simulink model "Digital_ACMC"  (R2026a)
settings: Solver=FixedStepAuto  StopTime=0.024  FixedStep=1e-8
undefined symbols (not defined in the file): Kbal, Ki_i, Ki_v, Kp_i, Kp_v, Vin
libraries: fl_lib x16, nesl_utility x11, ee_lib x4, eeGeneralControl x3, eePwmGenerator x2, simulink x1
settings Model: Creator=ardas  LastModifiedBy=ardas
settings SimscapeCC: SimscapeNominalValues="[{\"value\":\"1\",\"unit\":\"A\"},{\"value\":\"1\",\"unit\":\"bar\"},{\"value\":\"1\",\"unit\":\"cm^2\"},{\"value\":\"1\",\"unit\":\"cm^3/s\"},{\"value\":\"1\",\"unit\":\"kJ/kg\"},{\"value\":\"1\",\"unit\":\"kW\"},{\"value\":\"1\",\"unit\":\"l\"},{\"value\":\"1\",\"unit\":\"N\"},{\"value\":\"1\",\"unit\":\"N*m\"},{\"value\":\"1\",\"unit\":\"V\"}]"  SimscapeLogType=none  SimscapeLogDataHistory=5000.0

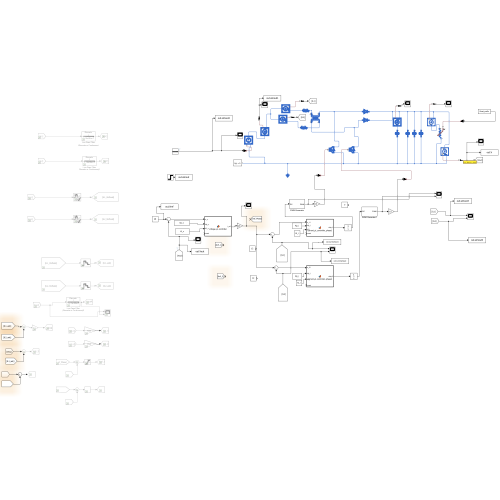
[thumbnail: Simulink's stored preview of the top-level diagram]
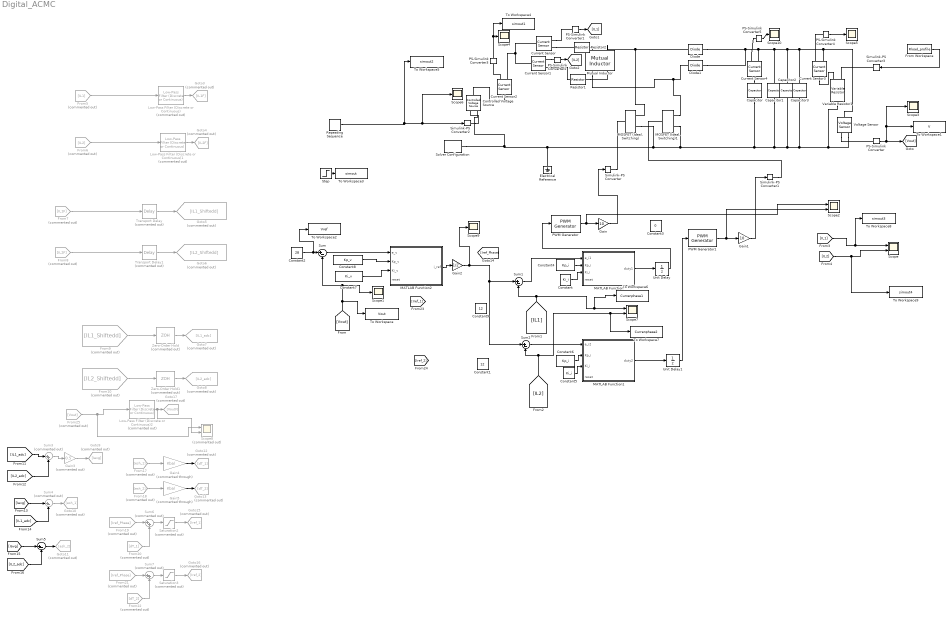
== system Digital_ACMC ==
  Capacitor : fl_lib/Electrical/Electrical Elements/Capacitor  c=330e-6 F  r=0.12 Ohm  g=0 1/Ohm  i_specify=off  i_priority=None  i=0 A  i_nominal_specify=off  i_nominal_value=1  i_nominal_unit=A  v_specify=off  v_priority=None  v=0 V  v_nominal_specify=off  v_nominal_value=1  v_nominal_unit=V  vc_specify=off  vc_priority=High  vc=0 V  vc_nominal_specify=off  vc_nominal_value=1  vc_nominal_unit=V
  Capacitor1 : fl_lib/Electrical/Electrical Elements/Capacitor  c=330e-6 F  r=0.12 Ohm  g=0 1/Ohm  i_specify=off  i_priority=None  i=0 A  i_nominal_specify=off  i_nominal_value=1  i_nominal_unit=A  v_specify=off  v_priority=None  v=0 V  v_nominal_specify=off  v_nominal_value=1  v_nominal_unit=V  vc_specify=off  vc_priority=High  vc=0 V  vc_nominal_specify=off  vc_nominal_value=1  vc_nominal_unit=V
  Capacitor2 : fl_lib/Electrical/Electrical Elements/Capacitor  c=47e-6 F  r=0.03 Ohm  g=0 1/Ohm  i_specify=off  i_priority=None  i=0 A  i_nominal_specify=off  i_nominal_value=1  i_nominal_unit=A  v_specify=off  v_priority=None  v=0 V  v_nominal_specify=off  v_nominal_value=1  v_nominal_unit=V  vc_specify=off  vc_priority=High  vc=0 V  vc_nominal_specify=off  vc_nominal_value=1  vc_nominal_unit=V
  Capacitor3 : fl_lib/Electrical/Electrical Elements/Capacitor  c=47e-6 F  r=0.03 Ohm  g=0 1/Ohm  i_specify=off  i_priority=None  i=0 A  i_nominal_specify=off  i_nominal_value=1  i_nominal_unit=A  v_specify=off  v_priority=None  v=0 V  v_nominal_specify=off  v_nominal_value=1  v_nominal_unit=V  vc_specify=off  vc_priority=High  vc=0 V  vc_nominal_specify=off  vc_nominal_value=1  vc_nominal_unit=V
  Constant : Constant  Value=Ki_i
  Constant1 : Constant  Value=12
  Constant2 : Constant  Value=28
  Constant3 : Constant  Value=0
  Constant4 : Constant  Value=Kp_i
  Constant5 : Constant  Value=Ki_i
  Constant6 : Constant  Value=Kp_i
  Constant7 : Constant  Value=Ki_v
  Constant8 : Constant  Value=Kp_v
  Constant9 : Constant  Value=12
  Controlled Voltage Source : fl_lib/Electrical/Electrical Sources/Controlled Voltage Source
  Current Sensor{,1..4} (5 alike) : fl_lib/Electrical/Electrical Sensors/Current Sensor
  Diode : ee_lib/Semiconductors & Converters/Diode  ModelType=ee.enum.diode.modelType.pwl  TableType=ee.enum.diode.tableType.IfMat  IfMat=[.07, .12, .19, 1.75, 4.24, 7.32, 11.2; .16, .3, .72, 2.14, 5.02, 8.35, 13.12] A  VfMat=[.9, 1.15, 1.25, 1.5, 1.75, 2.17, 2.6, 2.85; .58, .68, .75, 1.1, 1.38, 1.77, 2.27, 2.7] V  TjVec=[25, 125] degC  VfVec=[.5, .7, .9, 1.3, 1.7, 2.1, 2.5] V  IfVec=[.1, .2, .5, 1, 2, 4, 7, 10] A  IrMat=[1e-06, 2e-06, 5e-06, 1e-05, 2.5e-05, 5e-05, .0001; 2e-06, 5e-06, 1e-05, 4e-05, 8e-05, .0002, .0005] A  VrMat=[10, 100, 200, 250, 300, 325, 350; 10, 70, 160, 220, 270, 300, 320] V  VrVec=[10, 20, 40, 50, 70, 80, 100] V  IrVec=[1e-06, 2e-06, 5e-06, 1e-05, 2e-05, 5e-05, .0001] A  Vf=0.6 V  Ron=0.3 Ohm  Goff=1e-8 S  prmExp=ee.enum.diode.expParam.useTwo  I12=[.0137, .545] A  V12=[.6, .7] V  RS=0 Ohm  Tmeas=298.15 K  IS=1e-12 A  ec=1  I1=0.0137 A  V1=0.6 V  N_series=1  N_parallel=1  ZenerEnable=false  Rz=0.3 Ohm  BV=inf V  C_param=ee.enum.diode.capParam.fixed  CJ=0 pF  CJ0=5 pF  Vvec=[.1, 10, 100] V  Cvec=[3.5, 1, .4] pF  VJ=1 V  Mgrad=0.5  FC=0.5  Q_param=ee.enum.diode.recoveryParam.off  iRM=-7.15 A  iF=4 A  didt=-750 A/us  trr_factor=3  trr=115 ns  Qrr=150 nA*s  Vr=-600 V  Ls=150 nH  Erec=0.03 J  TT=50 ns  tau=100 ns  T_param=ee.enum.diode.temperatureParam.off  Tdevice=298.15 K  I1_T2=0.245 A  V1_T2=0.5 V  IS_T2=1.25e-7 A  Tmeas2=125 degC  XTI_param=ee.enum.diode.xtiParam.pn  XTI=3  EG_param=ee.enum.diode.egapParam.material_si  EG=1.11 eV  dBVdT=0 V/K  enable_fault_input=simscape.enum.onoff.off  i_specify=off  i_priority=None  i=0 A  i_nominal_specify=off  i_nominal_value=1  i_nominal_unit=A  v_specify=off  v_priority=None  v=0 V  v_nominal_specify=off  v_nominal_value=1  v_nominal_unit=V  v_capacitor_specify=off  v_capacitor_priority=None  v_capacitor=0 V  v_capacitor_nominal_specify=off  v_capacitor_nominal_value=1  v_capacitor_nominal_unit=V  Qj_specify=off  Qj_priority=High  Qj=0 C  Qj_nominal_specify=off  Qj_nominal_value=1  Qj_nominal_unit=C  i_diode_specify=off  i_diode_priority=None  i_diode=0 A  i_diode_nominal_specify=off  i_diode_nominal_value=1  i_diode_nominal_unit=A  v_diode_specify=off  v_diode_priority=None  v_diode=0 V  v_diode_nominal_specify=off  v_diode_nominal_value=1  v_diode_nominal_unit=V  i_capacitor_specify=off  i_capacitor_priority=None  i_capacitor=0 A  i_capacitor_nominal_specify=off  i_capacitor_nominal_value=1  i_capacitor_nominal_unit=A  fidelity_level=ee.enum.diode.fidelity.includeChargeDyn  rec_loss_model=ee.enum.diode.reverseRecoveryModel.fixed  ErecVal=0 J  scaleWithIandV=true  ErecMat=zeros(2, 3) J  ErecMat3D=zeros(2, 3, 2) J  TjrecVec=[298.15, 398.15] K  IfrecVec=[.1, 1, 10] A  IrecVal=10 A  VrecVal=10 V  VrecVec=[0, 100] V  tFilter=1 / 1000 / 100 s  thermal_network_parameterization=ee.enum.thermalNetworkTopology.junctionCase  Rth=[0, 10] K/W  Rth_Cauer=[1, 3, 10] K/W  Rth_Foster=[.08, .14, .22, .16] K/W  thermal_mass_parameterization=ee.enum.thermalNetwork.timeconstant  thermal_mass=[0, 1] J/K  thermal_mass_Cauer=[.1, .3, 1] J/K  thermal_mass_Foster=[.001, .005, .05, .5] J/K  thermal_time_constant=[0, 10] s  thermal_time_constant_Cauer=[1, 3, 10] s  thermal_time_constant_Foster=[7e-05, .0007, .01, .08] s  thermal_mass_initial_temperatures=[25, 25] degC  thermal_mass_initial_temperatures_Cauer=[25, 25, 25] degC  junction_thermal_mass=0.01 J/K  Tvec_initial_Foster=[25, 25, 25, 25] degC  no_thermal_network=0  junction_temperature_specify=off  junction_temperature_priority=None  junction_temperature=25 degC  junction_temperature_nominal_specify=off  junction_temperature_nominal_value=1  junction_temperature_nominal_unit=degC
  Diode1 : ee_lib/Semiconductors & Converters/Diode  ModelType=ee.enum.diode.modelType.pwl  TableType=ee.enum.diode.tableType.IfMat  IfMat=[.07, .12, .19, 1.75, 4.24, 7.32, 11.2; .16, .3, .72, 2.14, 5.02, 8.35, 13.12] A  VfMat=[.9, 1.15, 1.25, 1.5, 1.75, 2.17, 2.6, 2.85; .58, .68, .75, 1.1, 1.38, 1.77, 2.27, 2.7] V  TjVec=[25, 125] degC  VfVec=[.5, .7, .9, 1.3, 1.7, 2.1, 2.5] V  IfVec=[.1, .2, .5, 1, 2, 4, 7, 10] A  IrMat=[1e-06, 2e-06, 5e-06, 1e-05, 2.5e-05, 5e-05, .0001; 2e-06, 5e-06, 1e-05, 4e-05, 8e-05, .0002, .0005] A  VrMat=[10, 100, 200, 250, 300, 325, 350; 10, 70, 160, 220, 270, 300, 320] V  VrVec=[10, 20, 40, 50, 70, 80, 100] V  IrVec=[1e-06, 2e-06, 5e-06, 1e-05, 2e-05, 5e-05, .0001] A  Vf=0.6 V  Ron=0.3 Ohm  Goff=1e-8 S  prmExp=ee.enum.diode.expParam.useTwo  I12=[.0137, .545] A  V12=[.6, .7] V  RS=0 Ohm  Tmeas=298.15 K  IS=1e-12 A  ec=1  I1=0.0137 A  V1=0.6 V  N_series=1  N_parallel=1  ZenerEnable=false  Rz=0.3 Ohm  BV=inf V  C_param=ee.enum.diode.capParam.fixed  CJ=0 pF  CJ0=5 pF  Vvec=[.1, 10, 100] V  Cvec=[3.5, 1, .4] pF  VJ=1 V  Mgrad=0.5  FC=0.5  Q_param=ee.enum.diode.recoveryParam.off  iRM=-7.15 A  iF=4 A  didt=-750 A/us  trr_factor=3  trr=115 ns  Qrr=150 nA*s  Vr=-600 V  Ls=150 nH  Erec=0.03 J  TT=50 ns  tau=100 ns  T_param=ee.enum.diode.temperatureParam.off  Tdevice=298.15 K  I1_T2=0.245 A  V1_T2=0.5 V  IS_T2=1.25e-7 A  Tmeas2=125 degC  XTI_param=ee.enum.diode.xtiParam.pn  XTI=3  EG_param=ee.enum.diode.egapParam.material_si  EG=1.11 eV  dBVdT=0 V/K  enable_fault_input=simscape.enum.onoff.off  i_specify=off  i_priority=None  i=0 A  i_nominal_specify=off  i_nominal_value=1  i_nominal_unit=A  v_specify=off  v_priority=None  v=0 V  v_nominal_specify=off  v_nominal_value=1  v_nominal_unit=V  v_capacitor_specify=off  v_capacitor_priority=None  v_capacitor=0 V  v_capacitor_nominal_specify=off  v_capacitor_nominal_value=1  v_capacitor_nominal_unit=V  Qj_specify=off  Qj_priority=High  Qj=0 C  Qj_nominal_specify=off  Qj_nominal_value=1  Qj_nominal_unit=C  i_diode_specify=off  i_diode_priority=None  i_diode=0 A  i_diode_nominal_specify=off  i_diode_nominal_value=1  i_diode_nominal_unit=A  v_diode_specify=off  v_diode_priority=None  v_diode=0 V  v_diode_nominal_specify=off  v_diode_nominal_value=1  v_diode_nominal_unit=V  i_capacitor_specify=off  i_capacitor_priority=None  i_capacitor=0 A  i_capacitor_nominal_specify=off  i_capacitor_nominal_value=1  i_capacitor_nominal_unit=A  fidelity_level=ee.enum.diode.fidelity.includeChargeDyn  rec_loss_model=ee.enum.diode.reverseRecoveryModel.fixed  ErecVal=0 J  scaleWithIandV=true  ErecMat=zeros(2, 3) J  ErecMat3D=zeros(2, 3, 2) J  TjrecVec=[298.15, 398.15] K  IfrecVec=[.1, 1, 10] A  IrecVal=10 A  VrecVal=10 V  VrecVec=[0, 100] V  tFilter=1 / 1000 / 100 s  thermal_network_parameterization=ee.enum.thermalNetworkTopology.junctionCase  Rth=[0, 10] K/W  Rth_Cauer=[1, 3, 10] K/W  Rth_Foster=[.08, .14, .22, .16] K/W  thermal_mass_parameterization=ee.enum.thermalNetwork.timeconstant  thermal_mass=[0, 1] J/K  thermal_mass_Cauer=[.1, .3, 1] J/K  thermal_mass_Foster=[.001, .005, .05, .5] J/K  thermal_time_constant=[0, 10] s  thermal_time_constant_Cauer=[1, 3, 10] s  thermal_time_constant_Foster=[7e-05, .0007, .01, .08] s  thermal_mass_initial_temperatures=[25, 25] degC  thermal_mass_initial_temperatures_Cauer=[25, 25, 25] degC  junction_thermal_mass=0.01 J/K  Tvec_initial_Foster=[25, 25, 25, 25] degC  no_thermal_network=0  junction_temperature_specify=off  junction_temperature_priority=None  junction_temperature=25 degC  junction_temperature_nominal_specify=off  junction_temperature_nominal_value=1  junction_temperature_nominal_unit=degC
  Electrical Reference : fl_lib/Electrical/Electrical Elements/Electrical Reference
  From Workspace : FromWorkspace  VariableName=Rload_profile
  From10 : From  Commented=on  GotoTag=IL2_Shiftedd
  From17 : From  Commented=on  GotoTag=esh_1
  From18 : From  Commented=on  GotoTag=esh_2
  From19 : From  Commented=on  GotoTag=Iref_Phase
  From20 : From  Commented=on  GotoTag=dT_1
  From21 : From  Commented=on  GotoTag=Iref_Phase
  From22 : From  Commented=on  GotoTag=dT_2
  From25 : From  Commented=on  GotoTag=Vout
  From5 : From  Commented=on  GotoTag=IL1
  From6 : From  Commented=on  GotoTag=IL2
  From7 : From  Commented=on  GotoTag=IL1F
  From8 : From  Commented=on  GotoTag=IL2F
  From9 : From  Commented=on  GotoTag=IL1_Shiftedd
  Gain : Gain  Gain=10
  Gain1 : Gain  Gain=10
  Gain2 : Gain  Gain=1/2
  Gain3 : Gain  Commented=on  Gain=0.5
  Gain4 : Gain  Commented=through  Gain=Kbal
  Gain5 : Gain  Commented=through  Gain=Kbal
  Goto10 : Goto  Commented=on  GotoTag=esh_1
  Goto11 : Goto  Commented=on  GotoTag=esh_2
  Goto12 : Goto  Commented=on  GotoTag=dT_1
  Goto13 : Goto  Commented=on  GotoTag=dT_2
  Goto15 : Goto  Commented=on  GotoTag=Iref_1
  Goto16 : Goto  Commented=on  GotoTag=Iref_2
  Goto17 : Goto  Commented=on  GotoTag=VoutF
  Goto3 : Goto  Commented=on  GotoTag=IL1F
  Goto4 : Goto  Commented=on  GotoTag=IL2F
  Goto5 : Goto  Commented=on  GotoTag=IL1_Shiftedd
  Goto6 : Goto  Commented=on  GotoTag=IL2_Shiftedd
  Goto7 : Goto  Commented=on  GotoTag=IL1_adc
  Goto8 : Goto  Commented=on  GotoTag=IL2_adc
  Goto9 : Goto  Commented=on  GotoTag=Iavg
  Low-Pass Filter (Discrete or Continuous) : eeGeneralControl/Low-Pass Filter (Discrete or Continuous)  Commented=on  K=1  T=3.18e-5  B=inf  A=-inf  init_option=Inherited from block input  x0=0  Ts=-1
  Low-Pass Filter (Discrete or Continuous)1 : eeGeneralControl/Low-Pass Filter (Discrete or Continuous)  Commented=on  K=1  T=3.18e-5  B=inf  A=-inf  init_option=Inherited from block input  x0=0  Ts=-1
  Low-Pass Filter (Discrete or Continuous)2 : eeGeneralControl/Low-Pass Filter (Discrete or Continuous)  Commented=on  K=1  T=0.00003979  B=inf  A=-inf  init_option=Inherited from block input  x0=0  Ts=-1
  MATLAB Function : MATLAB Function  TreatAsAtomicUnit=on  SystemSampleTime=1e-5
  MATLAB Function1 : MATLAB Function  TreatAsAtomicUnit=on  SystemSampleTime=1e-5
  MATLAB Function2 : MATLAB Function  TreatAsAtomicUnit=on  SystemSampleTime=1e-4
  "MOSFET (Ideal, Switching)" : ee_lib/Semiconductors & Converters/MOSFET (Ideal, Switching)  port_option=ee.enum.controlport.ps  Rds=0.0028 Ohm  Goff=1e-6 1/Ohm  Vth=1.7 V  diode_param=ee.enum.semiconductors.protectionDiode.nodynamics  diode_Vf=0.83 V  diode_Ron=0.001 Ohm  diode_Goff=1e-5 1/Ohm  diode_C=50e-9 F  diode_iRM=-235 A  diode_iF=300 A  diode_idot=-50 A/us  diode_trr_param=ee.enum.converters.diodeReverseParam.trr_factor  diode_trr_factor=3  diode_trr=15 us  diode_Qrr=1500 s*uA  ids_specify=off  ids_priority=None  ids=0 A  ids_nominal_specify=off  ids_nominal_value=1  ids_nominal_unit=A  vds_specify=off  vds_priority=None  vds=0 V  vds_nominal_specify=off  vds_nominal_value=1  vds_nominal_unit=V  vgs_specify=off  vgs_priority=None  vgs=0 V  vgs_nominal_specify=off  vgs_nominal_value=1  vgs_nominal_unit=V  thermal_loss_option=ee.enum.converters.thermalLossOption.constantvalues  Von_data=[0, 1.8, 3.2, 6, 10, 16; 0, 2, 5.5, 9.5, 15, 25] V  Tj=[298.15, 448.15] K  Iout_data=[0, 20, 40, 60, 80, 100] A  tabulateWithVds=false  Eon_data=[0, 55.04, 124.57, 235.53, 362.12; 0, 71.25, 161.25, 304.88, 468.75] * 1e-6 J  Eoff_data=[0, 18, 30, 56.1, 76.5; 0, 22.5, 37.5, 70.13, 95.63] * 1e-6 J  Eon_data_3D=[zeros(2, 5, 3)] J  Eoff_data_3D=[zeros(2, 5, 3)] J  Tj_loss=[298.15, 448.15] K  Iout_data_loss=[0, 10, 20, 30, 40] A  Vds_loss=[0, 150, 300] V  Eon_scalar=22.86e-3 J  Eoff_scalar=17.14e-3 J  Voff=300 V  Iout_scalar=600 A  useCurrentFromPreviousCycle=false  useVoltageFromPreviousCycle=false  diodeModelType=ee.enum.converters.diodeModelType.pwl  diodeTableType=ee.enum.diode.tableType.IfMat  diode_ReverseIVType=ee.enum.diode.diodeReverseIV.constant  diode_IfMat=[.07, .12, .19, 1.75, 4.24, 7.32, 11.2; .16, .3, .72, 2.14, 4.02, 6.35, 9.12] A  diode_VfMat=[.9, 1.15, 1.25, 1.5, 1.75, 2.17, 2.6, 2.85; .58, .68, .75, 1.1, 1.38, 1.77, 2.27, 2.7] V  diode_TjVec=[25, 125] degC  diode_VfVec=[.5, .7, .9, 1.3, 1.7, 2.1, 2.5] V  diode_IfVec=[.1, .2, .5, 1, 2, 4, 7, 10] A  diode_IrMat=[1e-06, 2e-06, 5e-06, 1e-05, 2.5e-05, 5e-05, .0001; 2e-06, 5e-06, 1e-05, 4e-05, 8e-05, .0002, .0005] A  diode_VrMat=[10, 100, 200, 250, 300, 325, 350; 10, 70, 160, 220, 270, 300, 320] V  diode_VrVec=[10, 20, 40, 50, 70, 80, 100] V  diode_IrVec=[1e-06, 2e-06, 5e-06, 1e-05, 2e-05, 5e-05, .0001] A  diode_Vr=-600 V  diode_Ls=150 nH  diode_Erec=0.03 J  diode_rec_loss_model=ee.enum.diode.reverseRecoveryModel.fixed  diode_ErecVal=0 J  diode_scaleWithIandV=true  diode_ErecMat=zeros(2, 3) J  diodeErecMat3D=zeros(2, 3, 2) J  diode_TjrecVec=[298.15, 398.15] K  diode_IfrecVec=[.1, 1, 10] A  diodeVrecVec=[0, 100] V  diode_IrecVal=10 A  diode_VrecVal=10 V  diode_tFilter=1 / 1000 / 100 s  separateThermalPortForDiode=false  thermal_network_parameterization=ee.enum.thermalNetworkTopology.external  Rth=[.03, .2] K/W  Rth_Cauer=[.03, .1, .2] K/W  Rth_Foster=[.08, .14, .22, .16] K/W  thermal_mass_parameterization=ee.enum.thermalNetwork.timeconstant  thermal_mass=[3, 25] J/K  thermal_mass_Cauer=[3, 10, 25] J/K  thermal_mass_Foster=[.001, .005, .05, .5] J/K  thermal_time_constant=[.1, 5] s  thermal_time_constant_Cauer=[.1, 1, 5] s  thermal_time_constant_Foster=[7e-05, .0007, .01, .08] s  thermal_mass_initial_temperatures=[25, 25] degC  thermal_mass_initial_temperatures_Cauer=[25, 25, 25] degC  junction_thermal_mass=0.1 J/K  Tvec_initial_Foster=[25, 25, 25, 25] degC  RthDiode=[.03, .2] K/W  RthCauerDiode=[.03, .1, .2] K/W  RthFosterDiode=[.03, .2] K/W  thermalMassDiode=[3, 25] J/K  thermalMassCauerDiode=[3, 10, 25] J/K  thermalMassFosterDiode=[33, 50] J/K  thermalTauDiode=[.1, 5] s  thermalTauCauerDiode=[.1, 1, 5] s  thermalTauFosterDiode=[1, 10] s  thermalMassInitTempDiode=[25, 25] degC  thermalMassInitTempCauerDiode=[25, 25, 25] degC  junctionthermalMassDiode=0.1 J/K  TVecInitialFosterDiode=[25, 25, 25, 25] degC  no_thermal_network=0  mosfet_junction_temperature_specify=off  mosfet_junction_temperature_priority=None  mosfet_junction_temperature=25 degC  mosfet_junction_temperature_nominal_specify=off  mosfet_junction_temperature_nominal_value=1  mosfet_junction_temperature_nominal_unit=degC  diode_junction_temperature_specify=off  diode_junction_temperature_priority=None  diode_junction_temperature=25 degC  diode_junction_temperature_nominal_specify=off  diode_junction_temperature_nominal_value=1  diode_junction_temperature_nominal_unit=degC  Qj_specify=off  Qj_priority=None  Qj=0 W  Qj_nominal_specify=off  Qj_nominal_value=1  Qj_nominal_unit=W  accumulatedSwitchingLosses_specify=off  accumulatedSwitchingLosses_priority=None  accumulatedSwitchingLosses=0 J
  "MOSFET (Ideal, Switching)1" : ee_lib/Semiconductors & Converters/MOSFET (Ideal, Switching)  port_option=ee.enum.controlport.ps  Rds=0.0028 Ohm  Goff=1e-6 1/Ohm  Vth=1.7 V  diode_param=ee.enum.semiconductors.protectionDiode.nodynamics  diode_Vf=0.83 V  diode_Ron=0.001 Ohm  diode_Goff=1e-5 1/Ohm  diode_C=50e-9 F  diode_iRM=-235 A  diode_iF=300 A  diode_idot=-50 A/us  diode_trr_param=ee.enum.converters.diodeReverseParam.trr_factor  diode_trr_factor=3  diode_trr=15 us  diode_Qrr=1500 s*uA  ids_specify=off  ids_priority=None  ids=0 A  ids_nominal_specify=off  ids_nominal_value=1  ids_nominal_unit=A  vds_specify=off  vds_priority=None  vds=0 V  vds_nominal_specify=off  vds_nominal_value=1  vds_nominal_unit=V  vgs_specify=off  vgs_priority=None  vgs=0 V  vgs_nominal_specify=off  vgs_nominal_value=1  vgs_nominal_unit=V  thermal_loss_option=ee.enum.converters.thermalLossOption.constantvalues  Von_data=[0, 1.8, 3.2, 6, 10, 16; 0, 2, 5.5, 9.5, 15, 25] V  Tj=[298.15, 448.15] K  Iout_data=[0, 20, 40, 60, 80, 100] A  tabulateWithVds=false  Eon_data=[0, 55.04, 124.57, 235.53, 362.12; 0, 71.25, 161.25, 304.88, 468.75] * 1e-6 J  Eoff_data=[0, 18, 30, 56.1, 76.5; 0, 22.5, 37.5, 70.13, 95.63] * 1e-6 J  Eon_data_3D=[zeros(2, 5, 3)] J  Eoff_data_3D=[zeros(2, 5, 3)] J  Tj_loss=[298.15, 448.15] K  Iout_data_loss=[0, 10, 20, 30, 40] A  Vds_loss=[0, 150, 300] V  Eon_scalar=22.86e-3 J  Eoff_scalar=17.14e-3 J  Voff=300 V  Iout_scalar=600 A  useCurrentFromPreviousCycle=false  useVoltageFromPreviousCycle=false  diodeModelType=ee.enum.converters.diodeModelType.pwl  diodeTableType=ee.enum.diode.tableType.IfMat  diode_ReverseIVType=ee.enum.diode.diodeReverseIV.constant  diode_IfMat=[.07, .12, .19, 1.75, 4.24, 7.32, 11.2; .16, .3, .72, 2.14, 4.02, 6.35, 9.12] A  diode_VfMat=[.9, 1.15, 1.25, 1.5, 1.75, 2.17, 2.6, 2.85; .58, .68, .75, 1.1, 1.38, 1.77, 2.27, 2.7] V  diode_TjVec=[25, 125] degC  diode_VfVec=[.5, .7, .9, 1.3, 1.7, 2.1, 2.5] V  diode_IfVec=[.1, .2, .5, 1, 2, 4, 7, 10] A  diode_IrMat=[1e-06, 2e-06, 5e-06, 1e-05, 2.5e-05, 5e-05, .0001; 2e-06, 5e-06, 1e-05, 4e-05, 8e-05, .0002, .0005] A  diode_VrMat=[10, 100, 200, 250, 300, 325, 350; 10, 70, 160, 220, 270, 300, 320] V  diode_VrVec=[10, 20, 40, 50, 70, 80, 100] V  diode_IrVec=[1e-06, 2e-06, 5e-06, 1e-05, 2e-05, 5e-05, .0001] A  diode_Vr=-600 V  diode_Ls=150 nH  diode_Erec=0.03 J  diode_rec_loss_model=ee.enum.diode.reverseRecoveryModel.fixed  diode_ErecVal=0 J  diode_scaleWithIandV=true  diode_ErecMat=zeros(2, 3) J  diodeErecMat3D=zeros(2, 3, 2) J  diode_TjrecVec=[298.15, 398.15] K  diode_IfrecVec=[.1, 1, 10] A  diodeVrecVec=[0, 100] V  diode_IrecVal=10 A  diode_VrecVal=10 V  diode_tFilter=1 / 1000 / 100 s  separateThermalPortForDiode=false  thermal_network_parameterization=ee.enum.thermalNetworkTopology.external  Rth=[.03, .2] K/W  Rth_Cauer=[.03, .1, .2] K/W  Rth_Foster=[.08, .14, .22, .16] K/W  thermal_mass_parameterization=ee.enum.thermalNetwork.timeconstant  thermal_mass=[3, 25] J/K  thermal_mass_Cauer=[3, 10, 25] J/K  thermal_mass_Foster=[.001, .005, .05, .5] J/K  thermal_time_constant=[.1, 5] s  thermal_time_constant_Cauer=[.1, 1, 5] s  thermal_time_constant_Foster=[7e-05, .0007, .01, .08] s  thermal_mass_initial_temperatures=[25, 25] degC  thermal_mass_initial_temperatures_Cauer=[25, 25, 25] degC  junction_thermal_mass=0.1 J/K  Tvec_initial_Foster=[25, 25, 25, 25] degC  RthDiode=[.03, .2] K/W  RthCauerDiode=[.03, .1, .2] K/W  RthFosterDiode=[.03, .2] K/W  thermalMassDiode=[3, 25] J/K  thermalMassCauerDiode=[3, 10, 25] J/K  thermalMassFosterDiode=[33, 50] J/K  thermalTauDiode=[.1, 5] s  thermalTauCauerDiode=[.1, 1, 5] s  thermalTauFosterDiode=[1, 10] s  thermalMassInitTempDiode=[25, 25] degC  thermalMassInitTempCauerDiode=[25, 25, 25] degC  junctionthermalMassDiode=0.1 J/K  TVecInitialFosterDiode=[25, 25, 25, 25] degC  no_thermal_network=0  mosfet_junction_temperature_specify=off  mosfet_junction_temperature_priority=None  mosfet_junction_temperature=25 degC  mosfet_junction_temperature_nominal_specify=off  mosfet_junction_temperature_nominal_value=1  mosfet_junction_temperature_nominal_unit=degC  diode_junction_temperature_specify=off  diode_junction_temperature_priority=None  diode_junction_temperature=25 degC  diode_junction_temperature_nominal_specify=off  diode_junction_temperature_nominal_value=1  diode_junction_temperature_nominal_unit=degC  Qj_specify=off  Qj_priority=None  Qj=0 W  Qj_nominal_specify=off  Qj_nominal_value=1  Qj_nominal_unit=W  accumulatedSwitchingLosses_specify=off  accumulatedSwitchingLosses_priority=None  accumulatedSwitchingLosses=0 J
  Mutual Inductor : fl_lib/Electrical/Electrical Elements/Mutual Inductor  L1=120 uH  L2=120 uH  perfectCoupling=false  k=0.7  i1_specify=off  i1_priority=None  i1=0 A  i1_nominal_specify=off  i1_nominal_value=1  i1_nominal_unit=A  i2_specify=off  i2_priority=None  i2=0 A  i2_nominal_specify=off  i2_nominal_value=1  i2_nominal_unit=A  v1_specify=off  v1_priority=None  v1=0 V  v1_nominal_specify=off  v1_nominal_value=1  v1_nominal_unit=V  v2_specify=off  v2_priority=None  v2=0 V  v2_nominal_specify=off  v2_nominal_value=1  v2_nominal_unit=V
  PS-Simulink Converter : nesl_utility/PS-Simulink Converter  PhysicalDomain=network_engine_domain  SubClassName=ps_output  LeftPortType=input  RightPortType=output  PseudoPeriodic=off  Frequencies=[]  VectorFormat=inherit  Unit=V  AffineConversion=off
  PS-Simulink Converter1 : nesl_utility/PS-Simulink Converter  PhysicalDomain=network_engine_domain  SubClassName=ps_output  LeftPortType=input  RightPortType=output  PseudoPeriodic=off  Frequencies=[]  VectorFormat=inherit  Unit=A  AffineConversion=off
  PS-Simulink Converter2 : nesl_utility/PS-Simulink Converter  PhysicalDomain=network_engine_domain  SubClassName=ps_output  LeftPortType=input  RightPortType=output  PseudoPeriodic=off  Frequencies=[]  VectorFormat=inherit  Unit=A  AffineConversion=off
  PS-Simulink Converter3 : nesl_utility/PS-Simulink Converter  PhysicalDomain=network_engine_domain  SubClassName=ps_output  LeftPortType=input  RightPortType=output  PseudoPeriodic=off  Frequencies=[]  VectorFormat=inherit  Unit=inherit  AffineConversion=off
  PS-Simulink Converter4 : nesl_utility/PS-Simulink Converter  PhysicalDomain=network_engine_domain  SubClassName=ps_output  LeftPortType=input  RightPortType=output  PseudoPeriodic=off  Frequencies=[]  VectorFormat=inherit  Unit=inherit  AffineConversion=off
  PS-Simulink Converter5 : nesl_utility/PS-Simulink Converter  PhysicalDomain=network_engine_domain  SubClassName=ps_output  LeftPortType=input  RightPortType=output  PseudoPeriodic=off  Frequencies=[]  VectorFormat=inherit  Unit=inherit  AffineConversion=off
  PWM Generator : eePwmGenerator/PWM Generator  CarrCount=Up  Tper=10e-6  Tdelay=0  Ts=0.00000001
  PWM Generator1 : eePwmGenerator/PWM Generator  CarrCount=Up  Tper=10e-6  Tdelay=10e-6/2  Ts=0.00000001
  Repeating Sequence : simulink/Sources/Repeating Sequence  rep_seq_t="[0  6e-3 12e-3 18e-3 24e-3 ]"  rep_seq_y=[Vin Vin Vin Vin Vin]
  Resistor1 : fl_lib/Electrical/Electrical Elements/Resistor  R=0.01 Ohm  i_specify=off  i_priority=None  i=0 A  i_nominal_specify=off  i_nominal_value=1  i_nominal_unit=A  v_specify=off  v_priority=None  v=0 V  v_nominal_specify=off  v_nominal_value=1  v_nominal_unit=V
  Resistor2 : fl_lib/Electrical/Electrical Elements/Resistor  R=0.01 Ohm  i_specify=off  i_priority=None  i=0 A  i_nominal_specify=off  i_nominal_value=1  i_nominal_unit=A  v_specify=off  v_priority=None  v=0 V  v_nominal_specify=off  v_nominal_value=1  v_nominal_unit=V
  Saturation2 : Saturate  Commented=on  UpperLimit=15
  Saturation3 : Saturate  Commented=on  UpperLimit=15
  Scope : Scope  NumInputPorts=2
      settings: ActiveDisplayYMinimum=13.12118877178229  ActiveDisplayYMaximum=16.285901492217782
  Scope{1,3..6,9..10} (7 alike) : Scope
      Scope1 settings: ActiveDisplayYMinimum=27.996735188156986  ActiveDisplayYMaximum=28.000584839765885
      Scope10 settings: ActiveDisplayYMinimum=-21.021061924806343  ActiveDisplayYMaximum=8.27266243165029  DataLoggingVariableName=ScopeData10
      Scope3 settings: ActiveDisplayYMinimum=-3.5667585387126168  ActiveDisplayYMaximum=32.100857060330128  DataLoggingVariableName=ScopeData3
      Scope4 settings: ActiveDisplayYMinimum=25.497706773431442  ActiveDisplayYMaximum=29.783336297580011  DataLoggingVariableName=ScopeData4
      Scope5 settings: ActiveDisplayYMinimum=-12.32466223431901  ActiveDisplayYMaximum=-10.00882655979523  DataLoggingVariableName=ScopeData5
      Scope6 settings: ActiveDisplayYMinimum=10  ActiveDisplayYMaximum=30  DataLoggingVariableName=ScopeData6
      Scope9 settings: ActiveDisplayYMinimum=9.4576280676363549  ActiveDisplayYMaximum=13.640782053911529  DataLoggingVariableName=ScopeData9
  Scope2 : Scope  NumInputPorts=2
      settings: ActiveDisplayYMinimum=-0.05013738001407067  ActiveDisplayYMaximum=1.1748487112641266  DataLoggingVariableName=ScopeData2
  Scope7 : Scope  NumInputPorts=2
      settings: ActiveDisplayYMinimum=13.787058146219982  ActiveDisplayYMaximum=13.928836276625423  DataLoggingVariableName=ScopeData7
  Scope8 : Scope  Commented=on  NumInputPorts=2
      settings: ActiveDisplayYMinimum=5.4638907833296742  ActiveDisplayYMaximum=25.7507092946611  DataLoggingVariableName=ScopeData8
  Simulink-PS Converter : nesl_utility/Simulink-PS Converter  PhysicalDomain=network_engine_domain  SubClassName=ps_input  LeftPortType=input  RightPortType=output  PseudoPeriodic=off  Frequencies=[]  NoiseDistribution=none  NoiseParameters=[]  Unit=1  AffineConversion=off  FilteringAndDerivatives=provide  SimscapeFilterOrder=1  InputFilterTimeConstant=0.001  UdotUserProvided=0
  Simulink-PS Converter1 : nesl_utility/Simulink-PS Converter  PhysicalDomain=network_engine_domain  SubClassName=ps_input  LeftPortType=input  RightPortType=output  PseudoPeriodic=off  Frequencies=[]  NoiseDistribution=none  NoiseParameters=[]  Unit=1  AffineConversion=off  FilteringAndDerivatives=provide  SimscapeFilterOrder=1  InputFilterTimeConstant=0.001  UdotUserProvided=0
  Simulink-PS Converter2 : nesl_utility/Simulink-PS Converter  PhysicalDomain=network_engine_domain  SubClassName=ps_input  LeftPortType=input  RightPortType=output  PseudoPeriodic=off  Frequencies=[]  NoiseDistribution=none  NoiseParameters=[]  Unit=1  AffineConversion=off  FilteringAndDerivatives=provide  SimscapeFilterOrder=1  InputFilterTimeConstant=0.001  UdotUserProvided=0
  Simulink-PS Converter3 : nesl_utility/Simulink-PS Converter  PhysicalDomain=network_engine_domain  SubClassName=ps_input  LeftPortType=input  RightPortType=output  PseudoPeriodic=off  Frequencies=[]  NoiseDistribution=none  NoiseParameters=[]  Unit=Ohm  AffineConversion=off  FilteringAndDerivatives=provide  SimscapeFilterOrder=1  InputFilterTimeConstant=0.001  UdotUserProvided=0
  Solver Configuration : nesl_utility/Solver Configuration  PhysicalDomain=network_engine_domain  SubClassName=solver  LeftPortType=input  RightPortType=generic  Tones=[]  Harmonics=[]  SimulateNoise=off  Profile=off  UseLocalSampling=off  EnableSwitchedLinearOptims=on  FrequencyDomain=off  UseCCode=off  RelTol=0.001  AbsTol=0.001  MinStep=1e-09  ToWorkspace=off  RevertToSquareIcSolve=off  NumHomotopyIterations=100  PhasorMode=off  PhasorModeNumHarmonics=1  ConsistencySolver=NEWTON_XTOL_AFTER_FTOL  CanonicalOrdering=UNORDERED  OptimizeIntermediates=UNOPTIMIZED  IndexReductionMethod=DerivativeReplacement  DoDC=off  ResidualTolerance=1e-09  ConsistencyTolSource=GLOBAL  ConsistencyAbsTol=0.001  ConsistencyRelTol=0.001  ConsistencyTolFactor=0.001  UseLocalSolver=off  LocalSolverChoice=NE_BACKWARD_EULER_ADVANCER  ResolveIndetEquations=on  FunctionEvalNumThread=1  LocalSolverSampleTime=0.001  DoFixedCost=off  MaxNonlinIter=3  MaxModeIter=2  ComputeImpulses=off  ImpulseIterations=2  LinearAlgebra=auto  LinearAlgebraNumThread=0  EquationFormulation=NE_TIME_EF  DelaysMemoryBudget=1024  AutomaticFiltering=on  FilteringTimeConstant=0.001  PartitionStorageMethod=AS_NEEDED  PartitionMemoryBudget=1024  PartitionMethod=ROBUST  MultibodyUseLocalSolver=off  MultibodyLocalSolverChoice=ODE1  MultibodyLocalSolverSampleTime=0.001
  Step : Step  Time=0  FinalValue=28  SampleTime=0
  Sum{,1..2,5} (4 alike) : Sum  Inputs=|+-
  Sum3 : Sum  Commented=on  Inputs=|++
  Sum4 : Sum  Commented=on  Inputs=|+-
  Sum6 : Sum  Commented=on  Inputs=|++
  Sum7 : Sum  Commented=on  Inputs=|++
  To Workspace : ToWorkspace  VariableName=Vout  SaveFormat=Timeseries  SampleTime=-1
  To Workspace1 : ToWorkspace  VariableName=V  SaveFormat=Timeseries  SampleTime=-1
  To Workspace2 : ToWorkspace  VariableName=Vref  SaveFormat=Timeseries  SampleTime=-1
  To Workspace3 : ToWorkspace  VariableName=simout  SaveFormat=Timeseries  SampleTime=-1
  To Workspace4 : ToWorkspace  VariableName=simout1  SaveFormat=Timeseries  SampleTime=-1
  To Workspace5 : ToWorkspace  VariableName=simout2  SaveFormat=Timeseries  SampleTime=-1
  To Workspace6 : ToWorkspace  VariableName=Currenphase1  SaveFormat=Timeseries  SampleTime=-1
  To Workspace7 : ToWorkspace  VariableName=Currenphase2  SaveFormat=Timeseries  SampleTime=-1
  To Workspace8 : ToWorkspace  VariableName=simout3  SaveFormat=Timeseries  SampleTime=-1
  To Workspace9 : ToWorkspace  VariableName=simout4  SaveFormat=Timeseries  SampleTime=-1
  Transport Delay : TransportDelay  Commented=on  DelayTime=5e-6
  Transport Delay1 : TransportDelay  Commented=on  DelayTime=5e-6
  Unit Delay : UnitDelay  SampleTime=-1
  Unit Delay1 : UnitDelay  SampleTime=-1
  Variable Resistor1 : fl_lib/Electrical/Electrical Elements/Variable Resistor  Rmin=0 Ohm  thermalEnable=false  thermal_mass=1 J/K  i_specify=off  i_priority=None  i=0 A  i_nominal_specify=off  i_nominal_value=1  i_nominal_unit=A  v_specify=off  v_priority=None  v=0 V  v_nominal_specify=off  v_nominal_value=1  v_nominal_unit=V  T_specify=off  T_priority=None  T=300 K  T_nominal_specify=off  T_nominal_value=1  T_nominal_unit=K
  Voltage Sensor : fl_lib/Electrical/Electrical Sensors/Voltage Sensor
  Zero-Order Hold : ZeroOrderHold  Commented=on  SampleTime=1e-5
  Zero-Order Hold1 : ZeroOrderHold  Commented=on  SampleTime=1e-5
  wires:
  PWM Generator/1 -> Scope2/1, Gain/1
  Gain/1 -> Simulink-PS Converter/1
  PWM Generator1/1 -> Scope2/2, Gain1/1
  Gain1/1 -> Simulink-PS Converter1/1
  PS-Simulink Converter/1 -> Scope3/1, To Workspace1/1, [Vout]
  [Vout] -> Scope1/1, Sum/2, To Workspace/1
  Constant2/1 -> To Workspace2/1, Sum/1
  Sum1/1 -> MATLAB Function/1(e_i1)
  PS-Simulink Converter1/1 -> [IL1]
  PS-Simulink Converter2/1 -> [IL2]
  Sum2/1 -> MATLAB Function1/1(e_i2)
  [IL1] -> To Workspace8/1, Scope/1
  [IL2] -> To Workspace9/1, Scope/2
  [IL1] -> To Workspace6/1, Scope7/1, Sum1/2
  [IL2] -> To Workspace7/1, Scope7/2, Sum2/2
  From5/1 -> Low-Pass Filter (Discrete or Continuous)/1
  Low-Pass Filter (Discrete or Continuous)/1 -> Goto3/1
  From6/1 -> Low-Pass Filter (Discrete or Continuous)1/1
  Low-Pass Filter (Discrete or Continuous)1/1 -> Goto4/1
  From7/1 -> Transport Delay/1
  Transport Delay/1 -> Goto5/1
  Transport Delay1/1 -> Goto6/1
  From8/1 -> Transport Delay1/1
  From9/1 -> Zero-Order Hold/1
  Zero-Order Hold/1 -> Goto7/1
  Zero-Order Hold1/1 -> Goto8/1
  From10/1 -> Zero-Order Hold1/1
  [IL1_adc] -> Sum3/1
  [IL2_adc] -> Sum3/2
  Sum3/1 -> Gain3/1
  Gain3/1 -> Goto9/1
  [Iavg] -> Sum4/1
  [IL1_adc] -> Sum4/2
  Sum4/1 -> Goto10/1
  [IL2_adc] -> Sum5/2
  Sum5/1 -> Goto11/1
  [Iavg] -> Sum5/1
  From17/1 -> Gain4/1
  Gain4/1 -> Goto12/1
  From18/1 -> Gain5/1
  Gain5/1 -> Goto13/1
  From19/1 -> Sum6/1
  From20/1 -> Sum6/2
  Sum6/1 -> Saturation2/1
  From22/1 -> Sum7/2
  From21/1 -> Sum7/1
  Sum7/1 -> Saturation3/1
  Saturation2/1 -> Goto15/1
  Saturation3/1 -> Goto16/1
  PS-Simulink Converter3/1 -> To Workspace4/1, Scope4/1
  From25/1 -> Scope8/1, Low-Pass Filter (Discrete or Continuous)2/1
  Low-Pass Filter (Discrete or Continuous)2/1 -> Scope8/2, Goto17/1
  PS-Simulink Converter4/1 -> Scope5/1
  Repeating Sequence/1 -> To Workspace5/1, Scope6/1, Simulink-PS Converter2/1
  Sum/1 -> MATLAB Function2/1(e_v)
  MATLAB Function/1(duty1) -> Unit Delay/1
  Unit Delay/1 -> PWM Generator/1
  MATLAB Function1/1(duty2) -> Unit Delay1/1
  Unit Delay1/1 -> PWM Generator1/1
  Constant/1 -> MATLAB Function/3(Ki_i)
  Constant5/1 -> MATLAB Function1/3(Ki_i)
  Constant4/1 -> MATLAB Function/2(Kp_i)
  Constant6/1 -> MATLAB Function1/2(Kp_i)
  Constant7/1 -> MATLAB Function2/3(Ki_v)
  Constant8/1 -> MATLAB Function2/2(Kp_v)
  MATLAB Function2/1(i_ref) -> Gain2/1
  Gain2/1 -> Scope9/1, Sum2/1, Sum1/1
  Step/1 -> To Workspace3/1
  PS-Simulink Converter5/1 -> Scope10/1
  From Workspace/1 -> Simulink-PS Converter3/1
  connections:
  Current Sensor1/LConn1 -- Current Sensor2/RConn2 -- Current Sensor/LConn1
  Mutual Inductor/RConn2 -- "MOSFET (Ideal, Switching)"/RConn1 -- Diode/LConn1
  Diode/RConn1 -- Capacitor1/LConn1 -- Capacitor2/LConn1 -- Voltage Sensor/LConn1 -- Current Sensor3/RConn2 -- Capacitor3/LConn1 -- Current Sensor4/RConn2 -- Diode1/RConn1
  "MOSFET (Ideal, Switching)1"/RConn1 -- Mutual Inductor/LConn1 -- Diode1/LConn1
  Simulink-PS Converter/RConn1 -- "MOSFET (Ideal, Switching)"/LConn1
  Simulink-PS Converter1/RConn1 -- "MOSFET (Ideal, Switching)1"/LConn1
  Voltage Sensor/RConn1 -- PS-Simulink Converter/LConn1
  Resistor2/RConn1 -- Mutual Inductor/RConn1
  Current Sensor/RConn1 -- PS-Simulink Converter1/LConn1
  Current Sensor1/RConn1 -- PS-Simulink Converter2/LConn1
  Current Sensor1/RConn2 -- Resistor1/LConn1
  Current Sensor/RConn2 -- Resistor2/LConn1
  Current Sensor2/RConn1 -- PS-Simulink Converter3/LConn1
  "MOSFET (Ideal, Switching)"/RConn2 -- "MOSFET (Ideal, Switching)1"/RConn2 -- Variable Resistor1/RConn1 -- Voltage Sensor/RConn2 -- Capacitor3/RConn1 -- Capacitor2/RConn1 -- Capacitor1/RConn1 -- Capacitor/RConn1 -- Solver Configuration/RConn1 -- Controlled Voltage Source/RConn2 -- Electrical Reference/LConn1
  Current Sensor3/RConn1 -- PS-Simulink Converter4/LConn1
  Simulink-PS Converter2/RConn1 -- Controlled Voltage Source/RConn1
  Controlled Voltage Source/LConn1 -- Current Sensor2/LConn1
  Current Sensor4/LConn1 -- Capacitor/LConn1
  Current Sensor4/RConn1 -- PS-Simulink Converter5/LConn1
  Resistor1/RConn1 -- Mutual Inductor/LConn2
  Simulink-PS Converter3/RConn1 -- Variable Resistor1/LConn1
  Current Sensor3/LConn1 -- Variable Resistor1/LConn2

== matlab function Digital_ACMC/MATLAB Function1 ==
  data: e_i2 input; duty2 output; Kp_i input; Ki_i input; reset input
function duty2 = current_pi_controller_phase2(e_i2, Kp_i, Ki_i, reset)
%#codegen
% Faz-2 iç akım döngüsü PI
% Tustin (trapezoidal) integrasyon + clamping anti-windup

persistent int_i2 e_i2_prev

if isempty(int_i2)
    int_i2 = 0;
    e_i2_prev = 0;
end

if reset
    int_i2 = 0;
    e_i2_prev = 0;
end

Ts   = 1e-5;   % Dosyadaki akım PI sample time
uMin = 0.0;
uMax = 0.9;

% Tustin integratör aday değeri
int_candidate = int_i2 + (Ki_i * Ts / 2.0) * (e_i2 + e_i2_prev);

% Doyumsuz kontrol
u_unsat = Kp_i * e_i2 + int_candidate;

% Saturation
if u_unsat > uMax
    duty2 = uMax;
elseif u_unsat < uMin
    duty2 = uMin;
else
    duty2 = u_unsat;
end

% Clamping anti-windup
if (u_unsat > uMax && e_i2 > 0) || (u_unsat < uMin && e_i2 < 0)
    int_i2 = int_i2;
else
    int_i2 = int_candidate;
end

e_i2_prev = e_i2;

== matlab function Digital_ACMC/MATLAB Function ==
  data: e_i1 input; duty1 output; Kp_i input; Ki_i input; reset input
function duty1 = current_pi_controller_phase1(e_i1, Kp_i, Ki_i, reset)
%#codegen
% Faz-1 iç akım döngüsü PI
% Tustin (trapezoidal) integrasyon + clamping anti-windup

persistent int_i1 e_i1_prev

if isempty(int_i1)
    int_i1 = 0;
    e_i1_prev = 0;
end

if reset
    int_i1 = 0;
    e_i1_prev = 0;
end

Ts   = 1e-5;   % Dosyadaki akım PI sample time
uMin = 0.0;
uMax = 0.9;

% Tustin integratör aday değeri
int_candidate = int_i1 + (Ki_i * Ts / 2.0) * (e_i1 + e_i1_prev);

% Doyumsuz kontrol
u_unsat = Kp_i * e_i1 + int_candidate;

% Saturation
if u_unsat > uMax
    duty1 = uMax;
elseif u_unsat < uMin
    duty1 = uMin;
else
    duty1 = u_unsat;
end

% Clamping anti-windup
if (u_unsat > uMax && e_i1 > 0) || (u_unsat < uMin && e_i1 < 0)
    int_i1 = int_i1;
else
    int_i1 = int_candidate;
end

e_i1_prev = e_i1;

== matlab function Digital_ACMC/MATLAB Function2 ==
  data: e_v input; Kp_v input; i_ref output; Ki_v input; reset input
function i_ref = voltage_pi_controller(e_v, Kp_v, Ki_v, reset)
%#codegen
% Dış voltaj döngüsü PI
% Tustin (trapezoidal) + clamping anti-windup

persistent int_v e_v_prev

if isempty(int_v)
    int_v = 0.0;
    e_v_prev = 0.0;
end

if reset
    int_v = 0.0;
    e_v_prev = 0.0;
end

Ts   = 1e-4;
uMin = 0.0;
uMax = 40.0;

% Varsayılan çıkış (coder için güvenli)
%%i_ref = 0.0;

% Tustin integratör aday değeri
int_candidate = int_v + (Ki_v * Ts / 2.0) * (e_v + e_v_prev);

% Doyumsuz PI çıkışı
u_unsat = Kp_v * e_v + int_candidate;

% Saturation
if u_unsat > uMax
    i_ref = uMax;
elseif u_unsat < uMin
    i_ref = uMin;
else
    i_ref = u_unsat;
end

% Anti-windup (clamping)
if ~((u_unsat > uMax && e_v > 0.0) || (u_unsat < uMin && e_v < 0.0))
    int_v = int_candidate;
end

% State update
e_v_prev = e_v;

end
